simulink library "Model_DG_Synchronous_Generator"  (R2022b)
settings: Solver=VariableStepAuto  StartTime=0.0  StopTime=10.0  RelTol=1e-3
libraries: eeGeneralControl x11, simulink x6, slpidlib x4, spsPositiveSequencePLLDrivenLib x3, spsAC1AExcitationSystemLib x1, spsAC4AExcitationSystemLib x1, spsAC5AExcitationSystemLib x1, spsDC1AExcitationSystemLib x1, spsDC2AExcitationSystemLib x1, spsST1AExcitationSystemLib x1, spsST2AExcitationSystemLib x1, spsPLL3phLib x1
(part 1 of 2)
settings Model: Creator=winkens  LastModifiedBy=winkens
settings SolverCC: AlgebraicLoopSolver=TrustRegion
settings DebuggingCC: UnconnectedInputMsg=warning  UnconnectedOutputMsg=warning  UnconnectedLineMsg=warning  SFMachineParentedDataDiag=warning
settings ModelReferenceCC: EnableRefExpFcnMdlSchedulingChecks=on
settings RTWCC: DLArmComputeVersion=19.05

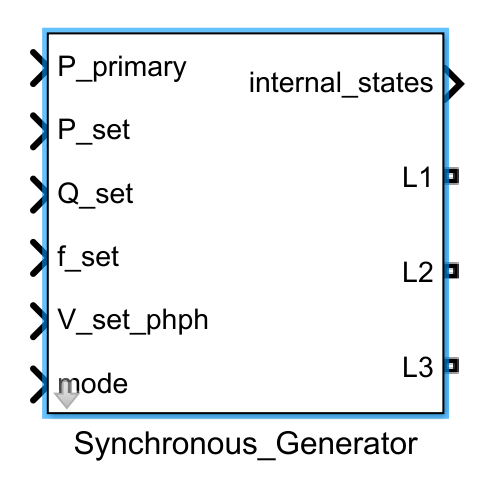
[thumbnail: Simulink's stored preview of the top-level diagram]
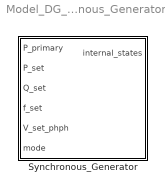
== system Model_DG_Synchronous_Generator ==
  Synchronous_Generator : Subsystem  mask{S_n=3.2e6, P_binst=2.0e6, V_n_phph=400, V_n_grid_phph=20e3, f_n=50, T_s_ctrl=1e-4, T_s_meas=1e-4, datatype='double', SG_Reactances=[ 3.19 0.33 0.159 1.79 0.155 0.05 ], SG_TimeConstants=[ 0.5 0.025 0.025 ], SG_StatorResistance=0.00074, SG_mech=[ 0.366 0.01 2 ], gov_type=IEEEG1 simplified, K_IEEEG1simp=10, T_IEEEG1simp=[ 0.2 0 0.1 0 ], dP_maxmin_IEEEG1simp=[ 2 -2 ], K_TGOV1=20, T_TGOV1=[ 0.2 0.6 2 ], kd_TGOV1=0.05, exciterModel=AC1A, QCtrl=Constant Voltage (no Q-Control), K_p_QCtrl=0.5, K_i_QCtrl=0.4, uq0ref=1.0, qmax=0.33, umax=1.04, deadband=0, p_pu=[0.1, 0.5, 0.6, 0.9, 1.0], q_pu=[0.0, 0.0, -0.05, -0.33, -0.33], p1=[0.94, 0.33], p2=[0.96, 0], p3=[1.04, 0], p4=[1.06, -0.33], cosphi_ref=1, ind_cap_Q=Inductive behavior (capacitive Q infeed), use_transformer=Grid coupling with transformer, RL_Trafo_GenSide=[ 0.002 0.08 ], RL_Trafo_GridSide=[ 0.002 0.08 ], Trafo_RmLm=[ 500 500 ]}
      mask prompts: S_n "Nominal Apparent Power [VA]"; P_binst "Installed Active Power [W]"; V_n_phph "Nominal Generator Voltage (rms, phase-to-phase) [V]"; V_n_grid_phph "Nominal Grid Voltage (rms, phase-to-phase) [V]"; f_n "Nominal Frequency [Hz]"; T_s_ctrl "Controller sample time [s]"; T_s_meas "Measurement sample time [s]"; datatype "Signal data type"; SG_Reactances "Reactances [ Xd Xd' Xd'' Xq Xq'' Xl ] (pu)"; SG_TimeConstants "Time constants [ Td' Td'' Tq'' ]  (s)"; SG_StatorResistance "Stator resistance (pu)"; SG_mech "Inertia, friction factor, pole pairs [ H(s) F(pu) p ]"; gov_type "Type"; K_IEEEG1simp "Droop Gain dP/df (pu)"; T_IEEEG1simp "Time Constants [ T1 T2 T3 T4 ] (s)"; dP_maxmin_IEEEG1simp "Max. rate of change of mech. power [ dP_max dP_min ] (pu)"; K_TGOV1 "Droop Gain dP/df (pu)"; T_TGOV1 "Time Constants [ T1 T2 T3 ] (s)"; kd_TGOV1 "Max. rate of change of mech. power [ dP_max dP_min ] (pu)"; exciterModel "Exciter Type"; QCtrl "Mode"; K_p_QCtrl "Q-Controller Proportional Gain"; K_i_QCtrl "Q-Controller Integral Gain"; uq0ref "U_Q0ref [pu]"; qmax "|Q_max| [pu]"; umax "U_max [pu]"; deadband "Voltage Deadband [+- %]"; p_pu "P_grid points [pu]"; q_pu "Q_grid points [pu]"; p1 "P1 [V_grid, Q_grid] [pu]"; p2 "P2 [V_grid, Q_grid] [pu]"; p3 "P3 [V_grid, Q_grid] [pu]"; p4 "P4 [V_grid, Q_grid] [pu]"; cosphi_ref "cos(phi)"; use_transformer "Transformer usage"; RL_Trafo_GenSide "SG-side winding impedance [ R L ] (pu):"; RL_Trafo_GridSide "Grid-side winding impedance [ R L ] (pu):"; Trafo_RmLm "Magnetization resistance and inductance [ Rm(pu) Lm(pu) ]"
      mask init:
      | alpha1 = (2*T_TGOV1(1)-T_s_ctrl) / (2*T_TGOV1(1)+T_s_ctrl);
      |     alpha2 = (2*T_TGOV1(2)-T_s_ctrl) / (2*T_TGOV1(2)+T_s_ctrl);
      |     alpha3 = (2*T_TGOV1(3)-T_s_ctrl) / (2*T_TGOV1(3)+T_s_ctrl);
      mask TypeOptions gov_type: IEEEG1 simplified | GAST (Generator Test Bench at Distribution Grid Laboratory) | TGOV1
      mask TypeOptions exciterModel: AC1A | AC4A | AC5A | DC1A | DC2A | ST1A | ST2A | AVR_Huette
      mask Callback exciterModel:
      | if strcmp(get_param(gcb,'exciterModel'),'AC1A')
      |     set_param([gcb '/SG_Control/Exciter'],'LabelModeActivechoice','AC1A');
      | 
      | elseif strcmp(get_param(gcb,'exciterModel'),'AC4A')
      |     set_param([gcb '/SG_Control/Exciter'],'LabelModeActivechoice','AC4A');
      | 
      | elseif strcmp(get_param(gcb,'exciterModel'),'AC5A')
      |     set_param([gcb '/SG_Control/Exciter'],'LabelModeActivechoice','AC5A');
      | 
      | elseif strcmp(get_param(gcb,'exciterModel'),'DC1A')
      |     set_param([gcb '/SG_Control/Exciter'],'LabelModeActivechoice','DC1A');
      | 
      | elseif strcmp(get_param(gcb,'exciterModel'),'DC2A')
      |     set_param([gcb '/SG_Control/Exciter'],'LabelModeActivechoice','DC2A');
      | 
      | elseif strcmp(get_param(gcb,'exciterModel'),'ST1A')
      |     set_param([gcb '/SG_Control/Exciter'],'LabelModeActivechoice','ST1A');
      | 
      | elseif strcmp(get_param(gcb,'exciterModel'),'ST2A')
      |     set_param([gcb '/SG_Control/Exciter'],'LabelModeActivechoice','ST2A');
      | 
      | elseif strcmp(get_param(gcb,'exciterModel'),'AVR_Huette')
      |     set_param([gcb '/SG_Control/Exciter'],'LabelModeActivechoice','AVR_Huette');
      | 
      | else
      |     set_param([gcb '/SG_Control/Exciter'],'LabelModeActivechoice','DC1A');
      | 
      | end
      mask TypeOptions QCtrl: Constant Voltage (no Q-Control) | Q(V)-Curve | Q(P)-Curve | Constant Q with Q(V)-Limitation | Constant cos(phi)
      mask Callback QCtrl:
      | msk = Simulink.Mask.get(gcb);
      | if strcmp(get_param(gcb,'QCtrl'),'Q(V)-Curve')
      |     %(a) Q(V)
      |     msk.getDialogControl('parambox_QV').Visible = 'on';
      |     msk.getDialogControl('parambox_QP').Visible = 'off';
      |     msk.getDialogControl('parambox_constQ').Visible = 'off';
      |     msk.getDialogControl('parambox_cosphi').Visible = 'off';
      | 
      | elseif strcmp(get_param(gcb,'QCtrl'),'Q(P)-Curve')
      |     %(b) Q(P)
      |     msk.getDialogControl('parambox_QV').Visible = 'off';
      |     msk.getDialogControl('parambox_QP').Visible = 'on';
      |     msk.getDialogControl('parambox_constQ').Visible = 'off';
      |     msk.getDialogControl('parambox_cosphi').Visible = 'off';
      | 
      | elseif strcmp(get_param(gcb,'QCtrl'),'Constant Q with Q(V)-Limitation')
      |     %(c) const Q
      |     msk.getDialogControl('parambox_QV').Visible = 'off';
      |     msk.getDialogControl('parambox_QP').Visible = 'off';
      |     msk.getDialogControl('parambox_constQ').Visible = 'on';
      |     msk.getDialogControl('parambox_cosphi').Visible = 'off';
      | 
      | elseif strcmp(get_param(gcb,'QCtrl'),'Constant cos(phi)')
      |     %(d) const cosphi
      |     msk.getDialogControl('parambox_QV').Visible = 'off';
      |     msk.getDialogControl('parambox_QP').Visible = 'off';
      |     msk.getDialogControl('parambox_constQ').Visible = 'off';
      |     msk.getDialogControl('parambox_cosphi').Visible = 'on';
      | 
      | elseif strcmp(get_param(gcb,'QCtrl'),'Constant Voltage (no Q-Control)')
      |     % no Q-Control
      |     msk.getDialogControl('parambox_QV').Visible = 'off';
      |     msk.getDialogControl('parambox_QP').Visible = 'off';
      |     msk.getDialogControl('parambox_constQ').Visible = 'off';
      |     msk.getDialogControl('parambox_cosphi').Visible = 'off';
      | 
      | end
      mask TypeOptions ind_cap_Q: Inductive behavior (capacitive Q infeed) | Capacitive behavior (inductive Q infeed)
      mask TypeOptions use_transformer: Direct grid coupling of SG (without transformer) | Grid coupling with transformer
      mask DialogControl DescGroupVar Prompt: Synchronous Generator
      mask DialogControl DescTextVar Prompt: Distributed generation unit using a synchronous generator for electromechanical energy conversion.
      mask DialogControl Container4 Prompt: General
      mask DialogControl Container24 Prompt: Sample Times and Data Types
      mask DialogControl Container5 Prompt: Synchr. Gen.
      mask DialogControl Control2 Prompt: All Synchronous Generator Parameters are defined in a per-unit-system based on the nominal apparent power, nominal generator voltage and nominal frequency defined in general-tab.
      mask DialogControl Container11 Prompt: Parameters
      mask DialogControl Container6 Prompt: Governor
      mask DialogControl Container13 Prompt: Parameters (Simplified IEEEG1-Governor-Turbine-Model)
      mask DialogControl Container13_copy Prompt: Parameters (TGOV1)
      mask DialogControl Container7 Prompt: Exciter
      mask DialogControl Container8 Prompt: Q-Control
      mask DialogControl Control3 Prompt: Reactive power control according to German MV grid codes VDE 4110. Choose constant voltage mode for no reactive power control in grid-forming units.
      mask DialogControl Container17 Prompt: Parameters
      mask DialogControl parambox_QV Prompt: Q(V) Parameters
      mask DialogControl parambox_QP Prompt: Q(P) Parameters
      mask DialogControl parambox_constQ Prompt: Constant Q with Q(V)-Limitation Parameters
      mask DialogControl parambox_cosphi Prompt: Constant cos(phi) Parameters
      mask DialogControl Container10 Prompt: Transformer
      mask DialogControl Control4 Prompt: Transformer parameters are defined in a per-unit-system based on the nominal power, the nominal frequency and the nominal voltages defined in tab General. The reference voltage for the impedance values depends on the respective nominal voltage level. However, magnetization resistance and inductance are based on the generator-side nominal voltage.
      mask DialogControl Container20 Prompt: Parameters

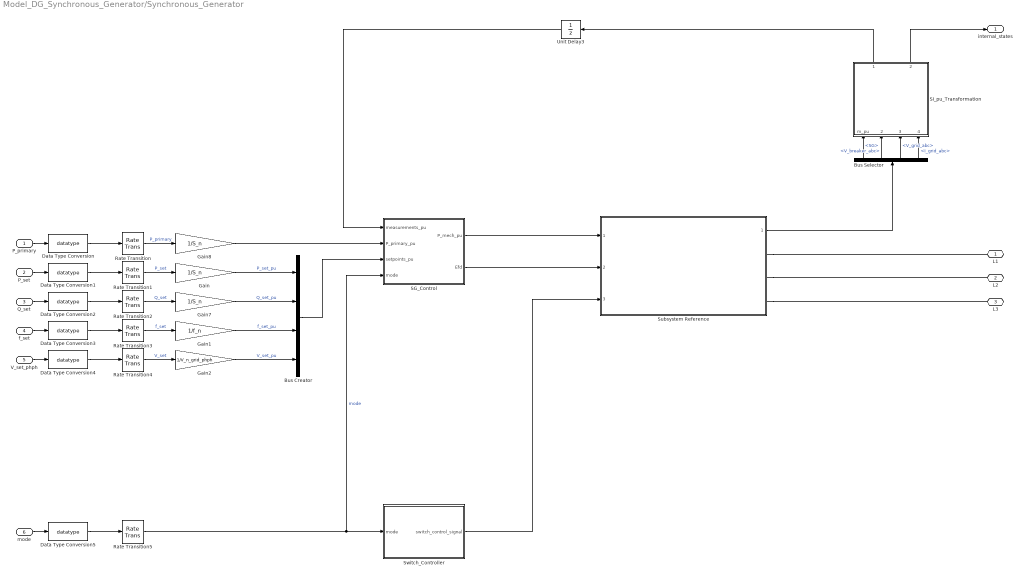
== system Model_DG_Synchronous_Generator/Synchronous_Generator ==
  P_primary : Inport
  P_set : Inport  Port=2
  Q_set : Inport  Port=3
  f_set : Inport  Port=4
  V_set_phph : Inport  Port=5
  mode : Inport  Port=6
  Bus Creator : BusCreator  Inputs=4
  Bus Selector : BusSelector  OutputSignals=SG,V_breaker_abc,V_grid_abc,I_grid_abc
  Data Type Conversion{,1..5} (6 alike) : DataTypeConversion  OutDataTypeStr=datatype  SaturateOnIntegerOverflow=off  RndMeth=Floor
  Gain : Gain  Gain=1/S_n
  Gain1 : Gain  Gain=1/f_n
  Gain2 : Gain  Gain=1/V_n_grid_phph
  Gain7 : Gain  Gain=1/S_n
  Gain8 : Gain  Gain=1/S_n
  Rate Transition{,1..5} (6 alike) : RateTransition  OutPortSampleTime=T_s_ctrl
  SG_Control : Subsystem
  SI_pu_Transformation : Subsystem
  Subsystem Reference : Subsystem  ReferencedSubsystem=Subsys_SG_Electromechanical_Part_SPS  S_n=S_n  f_n=f_n  V_n_phph=V_n_phph  V_n_grid_phph=V_n_grid_phph  SG_Reactances=SG_Reactances  SG_TimeConstants=SG_TimeConstants  SG_StatorResistance=SG_StatorResistance  SG_mech=SG_mech  use_transformer=use_transformer - 1  RL_Trafo_GenSide=RL_Trafo_GenSide  RL_Trafo_GridSide=RL_Trafo_GridSide  Rm_Lm=Trafo_RmLm  T_s_meas=T_s_meas  datatype=datatype
  Switch_Controller : Subsystem
  Unit Delay3 : UnitDelay  SampleTime=-1  HasFrameUpgradeWarning=on
  L1 : PMIOPort  Side=Right
  L2 : PMIOPort  Port=2  Side=Right
  L3 : PMIOPort  Port=3  Side=Right
  internal_states : Outport
  wires:
  V_set_phph/1 -> Data Type Conversion4/1
  P_set/1 -> Data Type Conversion1/1
  f_set/1 -> Data Type Conversion3/1
  SI_pu_Transformation/2(measurements_SI) -> internal_states/1
  SI_pu_Transformation/1(measurements_pu) -> Unit Delay3/1
  Q_set/1 -> Data Type Conversion2/1
  P_primary/1 -> Data Type Conversion/1
  Gain/1 -> Bus Creator/1  "P_set_pu"
  Gain7/1 -> Bus Creator/2  "Q_set_pu"
  Gain1/1 -> Bus Creator/3  "f_set_pu"
  Gain2/1 -> Bus Creator/4  "V_set_pu"
  SG_Control/1(P_mech_pu) -> Subsystem Reference/1
  SG_Control/2(Efd) -> Subsystem Reference/2
  Gain8/1 -> SG_Control/2(P_primary_pu)
  Bus Creator/1 -> SG_Control/3(setpoints_pu)
  Unit Delay3/1 -> SG_Control/1(measurements_pu)
  Data Type Conversion5/1 -> Rate Transition5/1
  Switch_Controller/1(switch_control_signal) -> Subsystem Reference/3
  Subsystem Reference/1 -> Bus Selector/1
  Bus Selector/1 -> SI_pu_Transformation/1(m_pu)  "<SG>"
  Bus Selector/2 -> SI_pu_Transformation/2(V_breaker_SI)  "<V_breaker_abc>"
  Bus Selector/3 -> SI_pu_Transformation/3(V_grid_SI)  "<V_grid_abc>"
  Bus Selector/4 -> SI_pu_Transformation/4(I_grid_SI)  "<I_grid_abc>"
  Data Type Conversion/1 -> Rate Transition/1
  Data Type Conversion1/1 -> Rate Transition1/1
  Data Type Conversion2/1 -> Rate Transition2/1
  Data Type Conversion3/1 -> Rate Transition3/1
  Data Type Conversion4/1 -> Rate Transition4/1
  mode/1 -> Data Type Conversion5/1
  Rate Transition/1 -> Gain8/1  "P_primary"
  Rate Transition1/1 -> Gain/1  "P_set"
  Rate Transition2/1 -> Gain7/1  "Q_set"
  Rate Transition3/1 -> Gain1/1  "f_set"
  Rate Transition4/1 -> Gain2/1  "V_set"
  Rate Transition5/1 -> SG_Control/4(mode), Switch_Controller/1(mode)  "mode"
  connections:
  Subsystem Reference/RConn2 -- L2/RConn1
  Subsystem Reference/RConn1 -- L1/RConn1
  Subsystem Reference/RConn3 -- L3/RConn1

== system Model_DG_Synchronous_Generator/Synchronous_Generator/SG_Control ==
  note: Speed Control
  note: Voltage Control
  note: Measurements and Setpoints
  measurements_pu : Inport
  P_primary_pu : Inport  Port=2
  setpoints_pu : Inport  Port=3
  mode : Inport  Port=4
  Bus Selector : BusSelector  OutputSignals="electrical_pu.V_breaker_rms_posSeq_pu,electrical_pu.V_grid_rms_posSeq_pu,SG_pu.Mechanical.Rotor speed  wm  (pu),electrical_pu.I_grid_pu,SG_pu.dq0 components.Field current  ifd (pu),electrical_pu.P_grid_pu,electrical_pu.Q_grid_pu,electrical_pu.V_grid_phase_posSeq,electrical_pu.V_breaker_phase_posSeq,electrical_pu.f_grid_PLL_pu"
  Bus Selector1 : BusSelector  OutputSignals=V_set_pu,f_set_pu,P_set_pu,Q_set_pu
  Exciter : Subsystem  Variant=on  VariantControlMode=label  LabelModeActiveChoice=AC1A
      settings: AttributesFormatString=%<BlockChoice>
  Governor_and_Turbine : Subsystem  Variant=on
  Multiport Switch : MultiPortSwitch  Inputs=2  DiagnosticForDefault=None  SaturateOnIntegerOverflow=off  InputSameDT=off
  Reactive_Power_Controller : Subsystem  Variant=on
  Synchronization_Controller : Subsystem
  P_mech_pu : Outport
  Efd : Outport  Port=2
  wires:
  Exciter/1(Efd) -> Efd/1
  Governor_and_Turbine/1(P_mech_pu) -> P_mech_pu/1
  Reactive_Power_Controller/1(V_stab_pu) -> Exciter/5(Vstab)
  measurements_pu/1 -> Bus Selector/1
  setpoints_pu/1 -> Bus Selector1/1
  Bus Selector1/3 -> Governor_and_Turbine/4(P_ref_pu)  "<P_set_pu>"
  Bus Selector/3 -> Governor_and_Turbine/3(omega_pu)  "<Rotor speed  wm  (pu)>"
  P_primary_pu/1 -> Governor_and_Turbine/5(P_primary_pu)
  Multiport Switch/1 -> Reactive_Power_Controller/2(V_grid_pu), Exciter/2(Vt)
  Bus Selector/4 -> Exciter/3(It)  "<I_grid_pu>"
  Bus Selector/5 -> Exciter/4(Ifd)  "<Field current  ifd (pu)>"
  mode/1 -> Multiport Switch/1, Governor_and_Turbine/1(mode), Reactive_Power_Controller/1(mode), Synchronization_Controller/1(mode)
  Bus Selector1/4 -> Reactive_Power_Controller/3(Q_set_pu)  "<Q_set_pu>"
  Bus Selector/2 -> Synchronization_Controller/4(V_grid_posSeq_pu), Multiport Switch/3  "<V_grid_rms_posSeq_pu>"
  Bus Selector/1 -> Multiport Switch/2  "<V_breaker_rms_posSeq_pu>"
  Bus Selector/6 -> Reactive_Power_Controller/4(P_grid_pu)  "<P_grid_pu>"
  Bus Selector/7 -> Reactive_Power_Controller/5(Q_grid_pu)  "<Q_grid_pu>"
  Synchronization_Controller/2(omega_ref_pu) -> Governor_and_Turbine/2(omega_ref_pu)
  Synchronization_Controller/1(V_ref_pu) -> Exciter/1(Vref)
  Bus Selector1/1 -> Synchronization_Controller/2(V_set_pu)  "<V_set_pu>"
  Bus Selector1/2 -> Synchronization_Controller/3(f_set_pu)  "<f_set_pu>"
  Bus Selector/8 -> Synchronization_Controller/5(theta_grid_posSeq)  "<V_grid_phase_posSeq>"
  Bus Selector/9 -> Synchronization_Controller/6(theta_breaker_posSeq)  "<V_breaker_phase_posSeq>"
  Bus Selector/10 -> Synchronization_Controller/7(f_grid_pu)  "<f_grid_PLL_pu>"

== system Model_DG_Synchronous_Generator/Synchronous_Generator/SI_pu_Transformation ==
  m_pu : Inport
  V_breaker_SI : Inport  Port=2
  V_grid_SI : Inport  Port=3
  I_grid_SI : Inport  Port=4
  Bus Creator : BusCreator  Inputs=11
  Bus Creator1 : BusCreator  Inputs=2
  Bus Creator2 : BusCreator  Inputs=2
  Electrical_Measurements_To_pu : Subsystem
  Positive_Sequence_Calculation : Subsystem
  SG_Measurements_To_SI : Subsystem
  measurements_pu : Outport
  measurements_SI : Outport  Port=2
  wires:
  m_pu/1 -> Bus Creator2/1, SG_Measurements_To_SI/1(m_pu)  "SG_pu"
  V_breaker_SI/1 -> Positive_Sequence_Calculation/2(V_breaker_abc), Bus Creator/1  "V_breaker_SI"
  V_grid_SI/1 -> Positive_Sequence_Calculation/1(V_grid_abc), Bus Creator/2  "V_grid_SI"
  I_grid_SI/1 -> Positive_Sequence_Calculation/3(I_grid_abc), Bus Creator/3  "I_grid_SI"
  Bus Creator/1 -> Bus Creator1/2, Electrical_Measurements_To_pu/1(el_SI)  "electrical_SI"
  Bus Creator1/1 -> measurements_SI/1
  Bus Creator2/1 -> measurements_pu/1
  Electrical_Measurements_To_pu/1(el_pu) -> Bus Creator2/2  "electrical_pu"
  SG_Measurements_To_SI/1(m_SI) -> Bus Creator1/1  "SG_SI"
  Positive_Sequence_Calculation/1(P_grid_SI) -> Bus Creator/4  "P_grid_SI"
  Positive_Sequence_Calculation/2(Q_grid_SI) -> Bus Creator/5  "Q_grid_SI"
  Positive_Sequence_Calculation/3(V_grid_rms_posSeq_SI) -> Bus Creator/6  "V_grid_rms_posSeq_SI"
  Positive_Sequence_Calculation/4(I_grid_rms_posSeq_SI) -> Bus Creator/7  "I_grid_rms_posSeq_SI"
  Positive_Sequence_Calculation/5(V_breaker_rms_posSeq_SI) -> Bus Creator/8  "V_breaker_rms_posSeq_SI"
  Positive_Sequence_Calculation/6(V_grid_phase_posSeq_SI) -> Bus Creator/9  "V_grid_phase_posSeq"
  Positive_Sequence_Calculation/7(V_breaker_phase_posSeq_SI) -> Bus Creator/10  "V_breaker_phase_posSeq"
  Positive_Sequence_Calculation/8(f_grid_PLL_SI) -> Bus Creator/11  "f_grid_PLL_SI"

== system Model_DG_Synchronous_Generator/Synchronous_Generator/Switch_Controller ==
  note: Blackstart
  note: Synchronization
  note: Grid Parallel Operation
  mode : Inport
  Constant{,1..3} (4 alike) : Constant
  Constant4 : Constant  Value=0
  Constant5 : Constant  Value=0
  Multiport Switch : MultiPortSwitch  DataPortOrder=Zero-based contiguous  zeroidx=on  SaturateOnIntegerOverflow=off  InputSameDT=off
  Mux : Mux  Inputs=2
  Mux1 : Mux  Inputs=2
  Mux2 : Mux  Inputs=2
  switch_control_signal : Outport
  wires:
  mode/1 -> Multiport Switch/1
  Multiport Switch/1 -> switch_control_signal/1
  Mux/1 -> Multiport Switch/2
  Mux2/1 -> Multiport Switch/4
  Mux1/1 -> Multiport Switch/3
  Constant/1 -> Mux/1
  Constant1/1 -> Mux/2
  Constant2/1 -> Mux2/1
  Constant3/1 -> Mux1/2
  Constant4/1 -> Mux1/1
  Constant5/1 -> Mux2/2

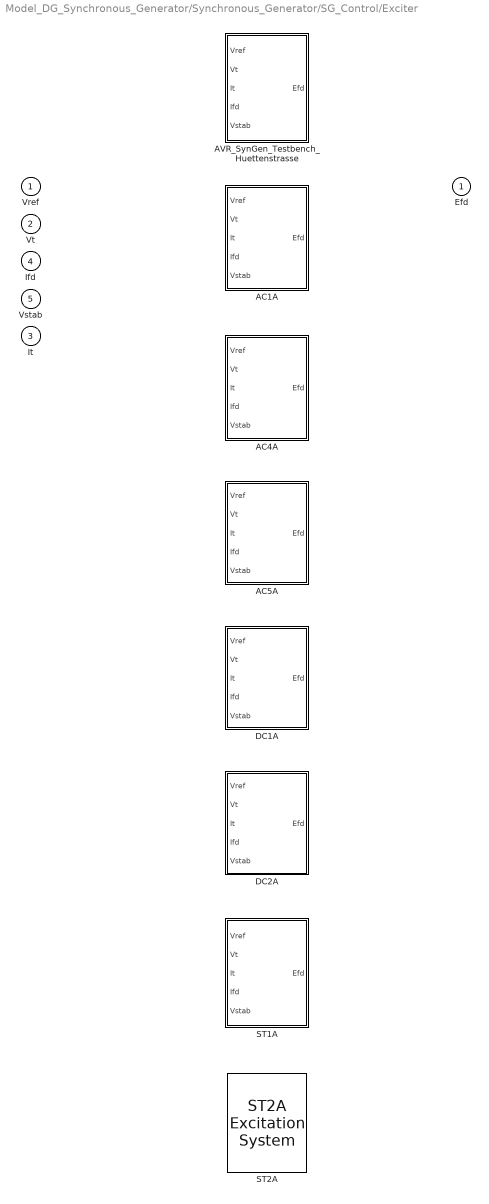
== system Model_DG_Synchronous_Generator/Synchronous_Generator/SG_Control/Exciter ==
  Vref : Inport
  Vt : Inport  Port=2
  It : Inport  Port=3
  Ifd : Inport  Port=4
  Vstab : Inport  Port=5
  AC1A : Subsystem  VariantControl=AC1A
  AC4A : Subsystem  VariantControl=AC4A
  AC5A : Subsystem  VariantControl=AC5A
  AVR_SynGen_Testbench_Huettenstrasse : Subsystem  VariantControl=AVR_Huette
  DC1A : Subsystem  VariantControl=DC1A
  DC2A : Subsystem  VariantControl=DC2A
  ST1A : Subsystem  VariantControl=ST1A
  ST2A : spsST2AExcitationSystemLib/ST2A Excitation System  VariantControl=ST2A  Tr=20e-3  KaTa=[120 0.15]  VRminmax=[0 1.0]  KfTf=[0.05 1.0]  KeTe=[1.0 0.5]  KI=0  Kp=4.88  Xd=1.56  Kc=0.1  v0=[1,1.42734]  I0=0.2739  TsBlock=-2
  Efd : Outport  VectorParamsAs1DForOutWhenUnconnected=off

== system Model_DG_Synchronous_Generator/Synchronous_Generator/SG_Control/Governor_and_Turbine ==
  note: 1) Add Subsystem or Model blocks as valid variant choices.
      | 2) You cannot connect blocks at this level. At simulation, connectivity is automatically
      | determined, based on the active variant and port name matching.
  mode : Inport
  omega_ref_pu : Inport  Port=2
  omega_pu : Inport  Port=3
  P_ref_pu : Inport  Port=4
  P_primary_pu : Inport  Port=5
  GAST_SyncGen_Testbench_Huettenstrasse : Subsystem  VariantControl=gov_type == 2
  IEEEG1_simplified : Subsystem  VariantControl=(default)
  TGOV1 : Subsystem  VariantControl=gov_type > 2.5
  P_mech_pu : Outport

== system Model_DG_Synchronous_Generator/Synchronous_Generator/SG_Control/Reactive_Power_Controller ==
  note: 1) Add Subsystem or Model blocks as valid variant choices.
      | 2) You cannot connect blocks at this level. At simulation, connectivity is automatically
      | determined, based on the active variant and port name matching.
  mode : Inport
  V_grid_pu : Inport  Port=2
  Q_set_pu : Inport  Port=3
  P_grid_pu : Inport  Port=4
  Q_grid_pu : Inport  Port=5
  Constant_Voltage : Subsystem  VariantControl=(default)
  Reactive_Power_Control : Subsystem  VariantControl=QCtrl > 1.5
  V_stab_pu : Outport

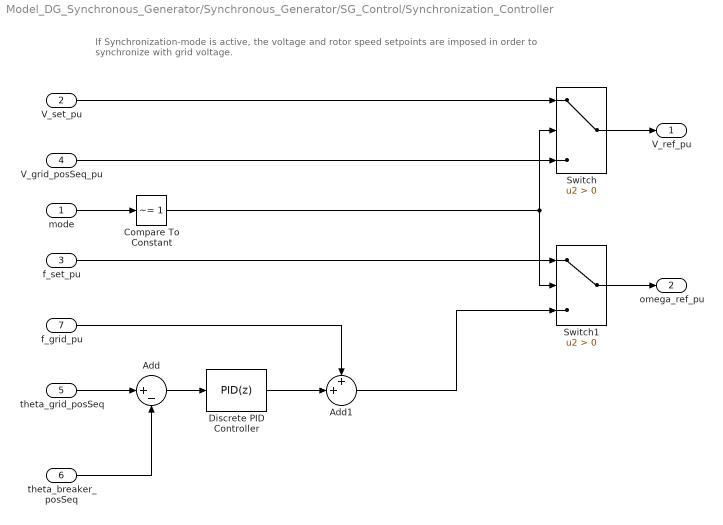
== system Model_DG_Synchronous_Generator/Synchronous_Generator/SG_Control/Synchronization_Controller ==
  note: If Synchronization-mode is active, the voltage and rotor speed setpoints are imposed in order to synchronize with grid voltage.
  mode : Inport
  V_set_pu : Inport  Port=2
  f_set_pu : Inport  Port=3
  V_grid_posSeq_pu : Inport  Port=4
  theta_grid_posSeq : Inport  Port=5
  theta_breaker_posSeq : Inport  Port=6
  f_grid_pu : Inport  Port=7
  Add : Sum  Inputs=|+-
  Add1 : Sum  Inputs=++|
  Compare To Constant : simulink/Logic and Bit Operations/Compare To Constant  relop=~=  const=1  OutDataTypeStr=boolean
  Discrete PID Controller : slpidlib/PID Controller  Controller=PID  Form=Parallel  TimeDomain=Discrete-time  UseExternalTs=off  SampleTime=-1  IntegratorMethod=Forward Euler  FilterMethod=Forward Euler  ControllerParametersSource=internal  P=0.01  I=0.01  UseKiTs=off  D=0.01  N=100  UseFilter=on  TunerSelectOption=Transfer Function Based (PID Tuner App)  InitialConditionSource=internal  InitialConditionForIntegrator=0  InitialConditionForFilter=0  DifferentiatorICPrevScaledInput=0  ExternalReset=none  TrackingMode=off  Kt=1  LimitOutput=on  SatLimitsSource=internal  UpperSaturationLimit=0.005  LowerSaturationLimit=-0.005  LinearizeAsGain=off  AntiWindupMode=clamping  Kb=1  LimitIntegrator=off  UpperIntegratorSaturationLimit=inf  LowerIntegratorSaturationLimit=-inf  POutMin=[]  POutMax=[]  IOutMin=[]  IOutMax=[]  DOutMin=[]  DOutMax=[]  NOutMin=[]  NOutMax=[]  SumOutMin=[]  SumOutMax=[]  SaturationOutMin=[]  SaturationOutMax=[]  PParamMin=[]  PParamMax=[]  IParamMin=[]  IParamMax=[]  DParamMin=[]  DParamMax=[]  NParamMin=[]  NParamMax=[]  KbParamMin=[]  KbParamMax=[]  KtParamMin=[]  KtParamMax=[]  KbOutMin=[]  KbOutMax=[]  KtOutMin=[]  KtOutMax=[]  IntegratorOutMin=[]  IntegratorOutMax=[]  FilterOutMin=[]  FilterOutMax=[]  SumI1OutMin=[]  SumI1OutMax=[]  SumI2OutMin=[]  SumI2OutMax=[]  SumI3OutMin=[]  SumI3OutMax=[]  SumI4OutMin=[]  SumI4OutMax=[]  SumDOutMin=[]  SumDOutMax=[]  DifferentiatorOutMin=[]  DifferentiatorOutMax=[]  FilterDiffOutCoefMin=[]  FilterDiffOutCoefMax=[]  ReciprocalOutMin=[]  ReciprocalOutMax=[]  SumDenOutMin=[]  SumDenOutMax=[]  SumNumOutMin=[]  SumNumOutMax=[]  DivideOutMin=[]  DivideOutMax=[]  UdiffTsProdOutMin=[]  UdiffTsProdOutMax=[]  NTsProdOutMin=[]  NTsProdOutMax=[]  UintegralTsProdOutMin=[]  UintegralTsProdOutMax=[]  UngainTsProdOutMin=[]  UngainTsProdOutMax=[]  ClampingZeroOutDataTypeStr=Inherit: Inherit via back propagation  ClampingZeroOutMin=[]  ClampingZeroOutMax=[]  FilterDenConstantOutDataTypeStr=Inherit: Inherit via back propagation  FilterDenConstantOutMin=[]  FilterDenConstantOutMax=[]  PCopyOutDataTypeStr=Inherit: Inherit via back propagation  PCopyOutMin=[]  PCopyOutMax=[]  NCopyOutDataTypeStr=Inherit: Inherit via back propagation  NCopyOutMin=[]  NCopyOutMax=[]  IntegratorContinuousStateAttributes=''  IntegratorStateMustResolveToSignalObject=off  IntegratorRTWStateStorageClass=Auto  FilterContinuousStateAttributes=''  FilterStateMustResolveToSignalObject=off  FilterRTWStateStorageClass=Auto  ParallelPVariant=InternalParameters  IdealPVariant=Disabled  IVariant=InternalParameters  DVariant=InternalParameters  IntegratorVariant=Discrete  SatVariant=Enabled  AWVariant=DiscClampingParallel  PCopyVariant=Disabled  TRVariant=Disabled  FdbkBlocksVariant=Forward  IdealPFdbkVariant=Disabled  SatFdbkVariant=Disabled  DerivativeFilterVariant=ForwardEulerFilter  NVariant=InternalParameters  NCopyVariant=Disabled  FilterICVariant=InternalICsFilter  IntegratorICVariant=InternalICs  ExternalResetVariant=Disabled  TRSumVariant=Passthrough  SumFdbkVariant=Disabled  SumVariant=Sum_PID  TsampFilterVariant=InternalTs  TsampNgainVariant=Passthrough  TsampIntegralVariant=Passthrough  ExternalSaturationOutDataTypeStr=Inherit: Same as second input
  Switch : Switch  Criteria=u2 > Threshold  SaturateOnIntegerOverflow=off  InputSameDT=off
  Switch1 : Switch  Criteria=u2 > Threshold  SaturateOnIntegerOverflow=off  InputSameDT=off
  V_ref_pu : Outport
  omega_ref_pu : Outport  Port=2
  wires:
  mode/1 -> Compare To Constant/1
  Switch/1 -> V_ref_pu/1
  Switch1/1 -> omega_ref_pu/1
  Compare To Constant/1 -> Switch/2, Switch1/2
  f_set_pu/1 -> Switch1/1
  V_set_pu/1 -> Switch/1
  V_grid_posSeq_pu/1 -> Switch/3
  theta_grid_posSeq/1 -> Add/1
  theta_breaker_posSeq/1 -> Add/2
  Add/1 -> Discrete PID Controller/1
  Discrete PID Controller/1 -> Add1/2
  Add1/1 -> Switch1/3
  f_grid_pu/1 -> Add1/1

== system Model_DG_Synchronous_Generator/Synchronous_Generator/SI_pu_Transformation/Electrical_Measurements_To_pu ==
  el_SI : Inport
  Bus Creator : BusCreator  Inputs=11
  Bus Selector : BusSelector  OutputSignals=V_breaker_SI,V_grid_SI,I_grid_SI,P_grid_SI,Q_grid_SI,V_grid_rms_posSeq_SI,I_grid_rms_posSeq_SI,V_breaker_rms_posSeq_SI,V_grid_phase_posSeq,V_breaker_phase_posSeq,f_grid_PLL_SI
  Gain{,1,5,7} (4 alike) : Gain  Gain=sqrt(3)/V_n_grid_phph
  Gain2 : Gain  Gain=(sqrt(3)*V_n_grid_phph) / S_n
  Gain3 : Gain  Gain=1/S_n
  Gain4 : Gain  Gain=1/S_n
  Gain6 : Gain  Gain=(sqrt(3)*V_n_grid_phph) / S_n
  Gain8 : Gain  Gain=1/f_n
  el_pu : Outport
  wires:
  el_SI/1 -> Bus Selector/1
  Bus Selector/1 -> Gain/1  "<V_breaker_SI>"
  Bus Selector/2 -> Gain1/1  "<V_grid_SI>"
  Bus Selector/3 -> Gain2/1  "<I_grid_SI>"
  Gain/1 -> Bus Creator/1  "V_breaker_pu"
  Gain1/1 -> Bus Creator/2  "V_grid_pu"
  Gain2/1 -> Bus Creator/3  "I_grid_pu"
  Bus Creator/1 -> el_pu/1
  Bus Selector/4 -> Gain3/1  "<P_grid_SI>"
  Gain3/1 -> Bus Creator/4  "P_grid_pu"
  Bus Selector/5 -> Gain4/1  "<Q_grid_SI>"
  Gain4/1 -> Bus Creator/5  "Q_grid_pu"
  Bus Selector/6 -> Gain5/1  "<V_grid_rms_posSeq_SI>"
  Gain5/1 -> Bus Creator/6  "V_grid_rms_posSeq_pu"
  Bus Selector/7 -> Gain6/1  "<I_grid_rms_posSeq_SI>"
  Gain6/1 -> Bus Creator/7  "I_grid_rms_posSeq_pu"
  Bus Selector/8 -> Gain7/1  "<V_breaker_rms_posSeq_SI>"
  Gain7/1 -> Bus Creator/8  "V_breaker_rms_posSeq_pu"
  Bus Selector/9 -> Bus Creator/9  "<V_grid_phase_posSeq>"
  Bus Selector/10 -> Bus Creator/10  "<V_breaker_phase_posSeq>"
  Bus Selector/11 -> Gain8/1  "<f_grid_PLL_SI>"
  Gain8/1 -> Bus Creator/11  "f_grid_PLL_pu"

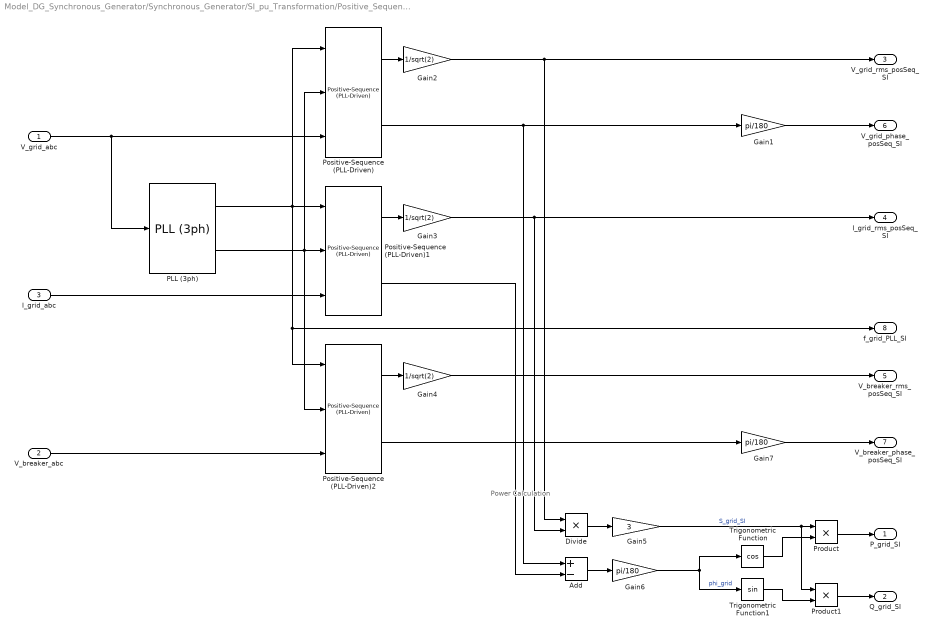
== system Model_DG_Synchronous_Generator/Synchronous_Generator/SI_pu_Transformation/Positive_Sequence_Calculation ==
  note: Power Calculation
  V_grid_abc : Inport
  V_breaker_abc : Inport  Port=2
  I_grid_abc : Inport  Port=3
  Add : Sum  Inputs=+-
  Divide : Product  Inputs=**
  Gain1 : Gain  Gain=pi/180
  Gain2 : Gain  Gain=1/sqrt(2)
  Gain3 : Gain  Gain=1/sqrt(2)
  Gain4 : Gain  Gain=1/sqrt(2)
  Gain5 : Gain  Gain=3
  Gain6 : Gain  Gain=pi/180
  Gain7 : Gain  Gain=pi/180
  PLL (3ph) : spsPLL3phLib/PLL (3ph)  Fmin=35  Par_Init=[0, 50]  ParK=[180, 3200, 1]  TcD=1e-4  MaxRateChangeFreq=12  FilterCutOffFreq=25  Ts=1e-4  AGC=on
  Positive-Sequence (PLL-Driven) : spsPositiveSequencePLLDrivenLib/Positive-Sequence (PLL-Driven)  Finit=50  Fmin=35  InInit=[0, 0]  Ts=T_s_meas
  Positive-Sequence (PLL-Driven)1 : spsPositiveSequencePLLDrivenLib/Positive-Sequence (PLL-Driven)  Finit=50  Fmin=35  InInit=[0, 0]  Ts=T_s_meas
  Positive-Sequence (PLL-Driven)2 : spsPositiveSequencePLLDrivenLib/Positive-Sequence (PLL-Driven)  Finit=50  Fmin=35  InInit=[0, 0]  Ts=T_s_meas
  Product : Product
  Product1 : Product
  Trigonometric Function : Trigonometry  Operator=cos
  Trigonometric Function1 : Trigonometry
  P_grid_SI : Outport
  Q_grid_SI : Outport  Port=2
  V_grid_rms_posSeq_SI : Outport  Port=3
  I_grid_rms_posSeq_SI : Outport  Port=4
  V_breaker_rms_posSeq_SI : Outport  Port=5
  V_grid_phase_posSeq_SI : Outport  Port=6
  V_breaker_phase_posSeq_SI : Outport  Port=7
  f_grid_PLL_SI : Outport  Port=8
  wires:
  V_grid_abc/1 -> PLL (3ph)/1, Positive-Sequence (PLL-Driven)/3
  I_grid_abc/1 -> Positive-Sequence (PLL-Driven)1/3
  V_breaker_abc/1 -> Positive-Sequence (PLL-Driven)2/3
  Positive-Sequence (PLL-Driven)2/1 -> Gain4/1
  Positive-Sequence (PLL-Driven)1/1 -> Gain3/1
  Positive-Sequence (PLL-Driven)/1 -> Gain2/1
  Gain2/1 -> Divide/1, V_grid_rms_posSeq_SI/1
  Gain3/1 -> Divide/2, I_grid_rms_posSeq_SI/1
  Gain4/1 -> V_breaker_rms_posSeq_SI/1
  Divide/1 -> Gain5/1
  Positive-Sequence (PLL-Driven)2/2 -> Gain7/1
  Gain5/1 -> Product1/1, Product/1  "S_grid_SI"
  Positive-Sequence (PLL-Driven)/2 -> Gain1/1, Add/1
  Positive-Sequence (PLL-Driven)1/2 -> Add/2
  Add/1 -> Gain6/1
  Gain6/1 -> Trigonometric Function1/1, Trigonometric Function/1  "phi_grid"
  Product1/1 -> Q_grid_SI/1
  Product/1 -> P_grid_SI/1
  Trigonometric Function/1 -> Product/2
  Trigonometric Function1/1 -> Product1/2
  PLL (3ph)/1 -> Positive-Sequence (PLL-Driven)2/1, f_grid_PLL_SI/1, Positive-Sequence (PLL-Driven)/1, Positive-Sequence (PLL-Driven)1/1
  PLL (3ph)/2 -> Positive-Sequence (PLL-Driven)/2, Positive-Sequence (PLL-Driven)2/2, Positive-Sequence (PLL-Driven)1/2
  Gain1/1 -> V_grid_phase_posSeq_SI/1
  Gain7/1 -> V_breaker_phase_posSeq_SI/1

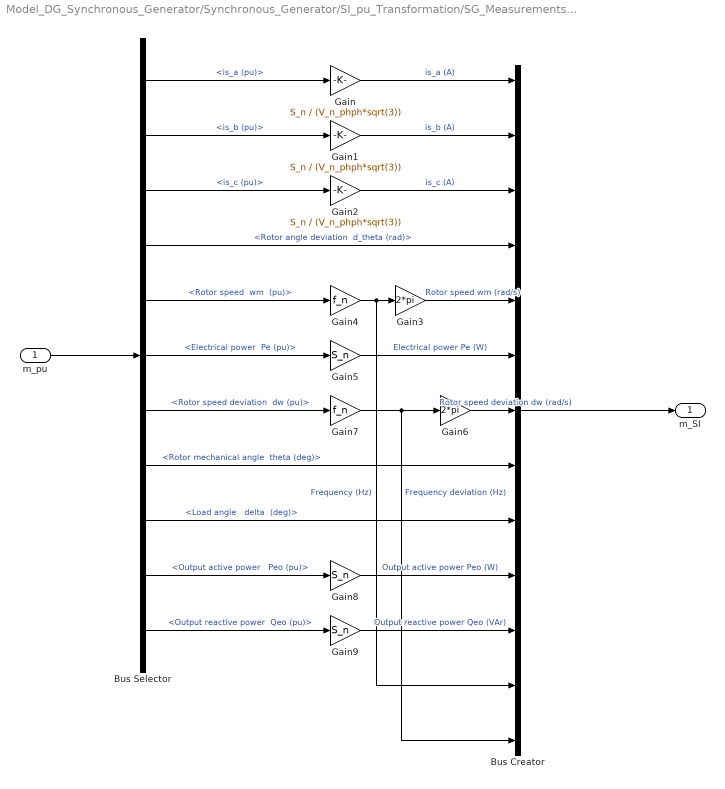
== system Model_DG_Synchronous_Generator/Synchronous_Generator/SI_pu_Transformation/SG_Measurements_To_SI ==
  m_pu : Inport
  Bus Creator : BusCreator  Inputs=13
  Bus Selector : BusSelector  OutputSignals="Stator current.is_a (pu),Stator current.is_b (pu),Stator current.is_c (pu),Mechanical.Rotor angle deviation  d_theta (rad),Mechanical.Rotor speed  wm  (pu),Mechanical.Electrical power  Pe (pu),Mechanical.Rotor speed deviation  dw (pu),Mechanical.Rotor mechanical angle  theta (deg),Load angle   delta  (deg),Output active power   Peo (pu),Output reactive power  Qeo (pu)"
  Gain : Gain  Gain=S_n / (V_n_phph*sqrt(3))
  Gain1 : Gain  Gain=S_n / (V_n_phph*sqrt(3))
  Gain2 : Gain  Gain=S_n / (V_n_phph*sqrt(3))
  Gain3 : Gain  Gain=2*pi
  Gain4 : Gain  Gain=f_n
  Gain5 : Gain  Gain=S_n
  Gain6 : Gain  Gain=2*pi
  Gain7 : Gain  Gain=f_n
  Gain8 : Gain  Gain=S_n
  Gain9 : Gain  Gain=S_n
  m_SI : Outport
  wires:
  m_pu/1 -> Bus Selector/1
  Bus Selector/1 -> Gain/1  "<is_a (pu)>"
  Bus Selector/2 -> Gain1/1  "<is_b (pu)>"
  Bus Selector/3 -> Gain2/1  "<is_c (pu)>"
  Bus Selector/4 -> Bus Creator/4  "<Rotor angle deviation  d_theta (rad)>"
  Bus Selector/5 -> Gain4/1  "<Rotor speed  wm  (pu)>"
  Gain4/1 -> Bus Creator/12, Gain3/1  "Frequency (Hz)"
  Gain3/1 -> Bus Creator/5  "Rotor speed wm (rad/s)"
  Bus Selector/6 -> Gain5/1  "<Electrical power  Pe (pu)>"
  Bus Selector/7 -> Gain7/1  "<Rotor speed deviation  dw (pu)>"
  Gain7/1 -> Gain6/1, Bus Creator/13  "Frequency deviation (Hz)"
  Gain6/1 -> Bus Creator/7  "Rotor speed deviation dw (rad/s)"
  Bus Selector/8 -> Bus Creator/8  "<Rotor mechanical angle  theta (deg)>"
  Bus Selector/9 -> Bus Creator/9  "<Load angle   delta  (deg)>"
  Bus Selector/10 -> Gain8/1  "<Output active power   Peo (pu)>"
  Bus Selector/11 -> Gain9/1  "<Output reactive power  Qeo (pu)>"
  Gain/1 -> Bus Creator/1  "is_a (A)"
  Gain1/1 -> Bus Creator/2  "is_b (A)"
  Gain2/1 -> Bus Creator/3  "is_c (A)"
  Gain5/1 -> Bus Creator/6  "Electrical power Pe (W)"
  Gain8/1 -> Bus Creator/10  "Output active power Peo (W)"
  Gain9/1 -> Bus Creator/11  "Output reactive power Qeo (VAr)"
  Bus Creator/1 -> m_SI/1

== system Model_DG_Synchronous_Generator/Synchronous_Generator/SG_Control/Exciter/AC1A ==
  Vref : Inport
  Vt : Inport  Port=2
  It : Inport  Port=3
  Ifd : Inport  Port=4
  Vstab : Inport  Port=5
  AC1A : spsAC1AExcitationSystemLib/AC1A Excitation System  Tr=20e-3  KaTa=[400 0.02]  VAminmax=[-14.5 14.5]  VRminmax=[-5.43 6.03]  KfTf=[0.03 1.0]  TbTc=[0 0]  KeTe=[1.0 0.80]  Ve12=[4.18 3.14]  SeVe12=[0.10 0.03]  Kd=0.38  Kc=0.20  v0=[0.000416667,0.000461832]*0  TsBlock=-2
  term3 : Terminator
  Efd : Outport  VectorParamsAs1DForOutWhenUnconnected=off
  wires:
  Vref/1 -> AC1A/1
  Vt/1 -> AC1A/2
  Ifd/1 -> AC1A/3
  Vstab/1 -> AC1A/4
  AC1A/1 -> Efd/1
  It/1 -> term3/1

== system Model_DG_Synchronous_Generator/Synchronous_Generator/SG_Control/Exciter/AC4A ==
  Vref : Inport
  Vt : Inport  Port=2
  It : Inport  Port=3
  Ifd : Inport  Port=4
  Vstab : Inport  Port=5
  AC4A : spsAC4AExcitationSystemLib/AC4A Excitation System  Tr=20e-3  KaTa=[200 0.015]  VIminmax=[-10 10]  VRminmax=[-4.53 5.64]  TbTc=[10 1.0]  Kc=0  v0=[1,1.42734]  TsBlock=-2
  term3 : Terminator
  Efd : Outport  VectorParamsAs1DForOutWhenUnconnected=off
  wires:
  Vref/1 -> AC4A/1
  Vt/1 -> AC4A/2
  Ifd/1 -> AC4A/3
  Vstab/1 -> AC4A/4
  AC4A/1 -> Efd/1
  It/1 -> term3/1

== system Model_DG_Synchronous_Generator/Synchronous_Generator/SG_Control/Exciter/AC5A ==
  Vref : Inport
  Vt : Inport  Port=2
  It : Inport  Port=3
  Ifd : Inport  Port=4
  Vstab : Inport  Port=5
  AC5A : spsAC5AExcitationSystemLib/AC5A Excitation System  Tr=20e-3  KaTa=[100 0.02]  VRminmax=[-7.3 7.3]  KfTf=[0.03 1 0 0]  KeTe=[1.0 0.8]  Efd12=[5.6 0.75*5.6]  SeEfd12=[0.86 0.5]  v0=[1,1.42734]  TsBlock=-2
  term3 : Terminator
  term4 : Terminator
  Efd : Outport  VectorParamsAs1DForOutWhenUnconnected=off
  wires:
  Vref/1 -> AC5A/1
  Vt/1 -> AC5A/2
  Vstab/1 -> AC5A/3
  AC5A/1 -> Efd/1
  It/1 -> term3/1
  Ifd/1 -> term4/1

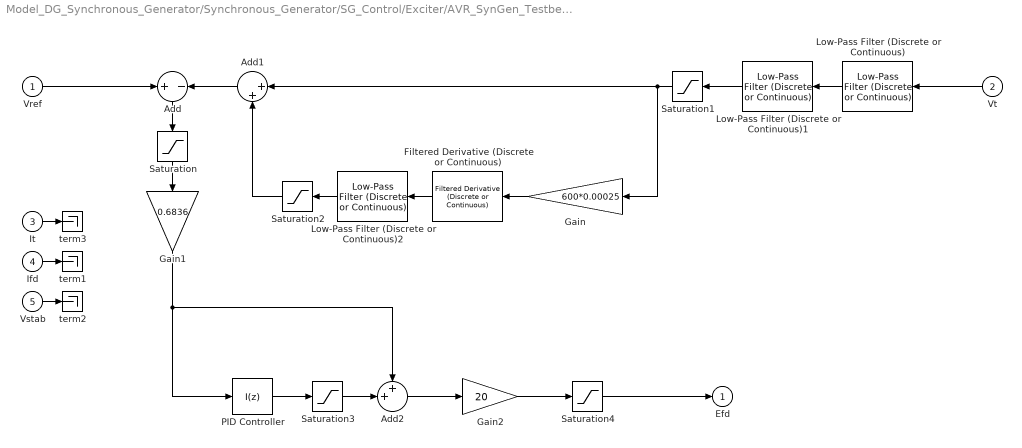
== system Model_DG_Synchronous_Generator/Synchronous_Generator/SG_Control/Exciter/AVR_SynGen_Testbench_Huettenstrasse ==
  Vref : Inport
  Vt : Inport  Port=2
  It : Inport  Port=3
  Ifd : Inport  Port=4
  Vstab : Inport  Port=5
  Add : Sum  Inputs=+|-
  Add1 : Sum  Inputs=|++
  Add2 : Sum  Inputs=++|
  Filtered Derivative (Discrete or Continuous) : eeGeneralControl/Filtered Derivative (Discrete or Continuous)  K=1  T=0.004  B=inf  A=-inf  minRatio=10  init_option=Inherited from block input  x0=0  Ts=-1
  Gain : Gain  Gain=600*0.00025
  Gain1 : Gain  Gain=0.6836
  Gain2 : Gain  Gain=20
  Low-Pass Filter (Discrete or Continuous) : eeGeneralControl/Low-Pass Filter (Discrete or Continuous)  K=1  T=0.002  B=inf  A=-inf  init_option=Inherited from block input  x0=0  Ts=-1
  Low-Pass Filter (Discrete or Continuous)1 : eeGeneralControl/Low-Pass Filter (Discrete or Continuous)  K=1  T=0.0005  B=inf  A=-inf  init_option=Inherited from block input  x0=0  Ts=-1
  Low-Pass Filter (Discrete or Continuous)2 : eeGeneralControl/Low-Pass Filter (Discrete or Continuous)  K=1  T=0.015  B=inf  A=-inf  init_option=Inherited from block input  x0=0  Ts=-1
  PID Controller : slpidlib/PID Controller  Controller=I  Form=Parallel  TimeDomain=Discrete-time  UseExternalTs=off  SampleTime=-1  IntegratorMethod=Forward Euler  FilterMethod=Forward Euler  ControllerParametersSource=internal  P=1  I=1200/131.072  D=0  UseFilter=on  N=100  TunerSelectOption=Transfer Function Based (PID Tuner App)  InitialConditionSource=internal  InitialConditionForIntegrator=0  InitialConditionForFilter=0  DifferentiatorICPrevScaledInput=0  ExternalReset=none  TrackingMode=off  Kt=1  LimitOutput=off  SatLimitsSource=internal  UpperSaturationLimit=inf  LowerSaturationLimit=-inf  LinearizeAsGain=on  AntiWindupMode=none  Kb=1  POutMin=[]  POutMax=[]  IOutMin=[]  IOutMax=[]  DOutMin=[]  DOutMax=[]  NOutMin=[]  NOutMax=[]  SumOutMin=[]  SumOutMax=[]  SaturationOutMin=[]  SaturationOutMax=[]  PParamMin=[]  PParamMax=[]  IParamMin=[]  IParamMax=[]  DParamMin=[]  DParamMax=[]  NParamMin=[]  NParamMax=[]  KbParamMin=[]  KbParamMax=[]  KtParamMin=[]  KtParamMax=[]  KbOutMin=[]  KbOutMax=[]  KtOutMin=[]  KtOutMax=[]  IntegratorOutMin=[]  IntegratorOutMax=[]  FilterOutMin=[]  FilterOutMax=[]  SumI1OutMin=[]  SumI1OutMax=[]  SumI2OutMin=[]  SumI2OutMax=[]  SumI3OutMin=[]  SumI3OutMax=[]  SumI4OutMin=[]  SumI4OutMax=[]  SumDOutMin=[]  SumDOutMax=[]  DifferentiatorOutMin=[]  DifferentiatorOutMax=[]  FilterDiffOutCoefMin=[]  FilterDiffOutCoefMax=[]  ReciprocalOutMin=[]  ReciprocalOutMax=[]  SumDenOutMin=[]  SumDenOutMax=[]  SumNumOutMin=[]  SumNumOutMax=[]  DivideOutMin=[]  DivideOutMax=[]  UdiffTsProdOutMin=[]  UdiffTsProdOutMax=[]  NTsProdOutMin=[]  NTsProdOutMax=[]  UintegralTsProdOutMin=[]  UintegralTsProdOutMax=[]  UngainTsProdOutMin=[]  UngainTsProdOutMax=[]  IntegratorContinuousStateAttributes=''  IntegratorStateMustResolveToSignalObject=off  IntegratorRTWStateStorageClass=Auto  FilterContinuousStateAttributes=''  FilterStateMustResolveToSignalObject=off  FilterRTWStateStorageClass=Auto  ParallelPVariant=Disabled  IdealPVariant=Disabled  IVariant=InternalParameters  DVariant=Disabled  IntegratorVariant=Discrete  SatVariant=Disabled  AWVariant=Passthrough  PCopyVariant=Disabled  TRVariant=Disabled  FdbkBlocksVariant=Forward  IdealPFdbkVariant=Disabled  SatFdbkVariant=Disabled  DerivativeFilterVariant=Disabled  NVariant=Disabled  NCopyVariant=Disabled_SignalSpec  FilterICVariant=Disabled  IntegratorICVariant=InternalICs  ExternalResetVariant=Disabled  TRSumVariant=Passthrough  SumFdbkVariant=Disabled  SumVariant=Passthrough_I  TsampFilterVariant=InternalTs  TsampNgainVariant=Passthrough  TsampIntegralVariant=Passthrough  ExternalSaturationOutDataTypeStr=Inherit: Same as second input
  Saturation : Saturate  UpperLimit=707  LowerLimit=-707
  Saturation1 : Saturate  UpperLimit=707  LowerLimit=-707
  Saturation2 : Saturate  UpperLimit=707  LowerLimit=-707
  Saturation3 : Saturate  UpperLimit=1418  LowerLimit=-1418
  Saturation4 : Saturate  UpperLimit=250  LowerLimit=-250
  term1 : Terminator
  term2 : Terminator
  term3 : Terminator
  Efd : Outport  VectorParamsAs1DForOutWhenUnconnected=off
  wires:
  It/1 -> term3/1
  Vt/1 -> Low-Pass Filter (Discrete or Continuous)/1
  Vref/1 -> Add/1
  Ifd/1 -> term1/1
  Vstab/1 -> term2/1
  Saturation4/1 -> Efd/1
  Add/1 -> Saturation/1
  Low-Pass Filter (Discrete or Continuous)/1 -> Low-Pass Filter (Discrete or Continuous)1/1
  Low-Pass Filter (Discrete or Continuous)1/1 -> Saturation1/1
  Add1/1 -> Add/2
  Saturation1/1 -> Gain/1, Add1/1
  Filtered Derivative (Discrete or Continuous)/1 -> Low-Pass Filter (Discrete or Continuous)2/1
  Gain/1 -> Filtered Derivative (Discrete or Continuous)/1
  Low-Pass Filter (Discrete or Continuous)2/1 -> Saturation2/1
  Saturation2/1 -> Add1/2
  Saturation/1 -> Gain1/1
  Gain1/1 -> Add2/1, PID Controller/1
  PID Controller/1 -> Saturation3/1
  Saturation3/1 -> Add2/2
  Add2/1 -> Gain2/1
  Gain2/1 -> Saturation4/1

== system Model_DG_Synchronous_Generator/Synchronous_Generator/SG_Control/Exciter/DC1A ==
  Vref : Inport
  Vt : Inport  Port=2
  It : Inport  Port=3
  Ifd : Inport  Port=4
  Vstab : Inport  Port=5
  DC1A : spsDC1AExcitationSystemLib/DC1A Excitation System  Tr=20e-3  KaTa=[46 0.06]  VRminmax=[-0.9 1.0]  KfTf=[0.1 1]  TbTc=[0 0]  KeTe=[0.05 0.46]  Efd12=[3.1 2.3]  SeEfd12=[0.33 0.10]  v0=[1,1.42734]  TsBlock=-2
  term3 : Terminator
  term4 : Terminator
  Efd : Outport  VectorParamsAs1DForOutWhenUnconnected=off
  wires:
  Vref/1 -> DC1A/1
  Vt/1 -> DC1A/2
  Vstab/1 -> DC1A/3
  DC1A/1 -> Efd/1
  It/1 -> term3/1
  Ifd/1 -> term4/1

== system Model_DG_Synchronous_Generator/Synchronous_Generator/SG_Control/Exciter/DC2A ==
  Vref : Inport
  Vt : Inport  Port=2
  It : Inport  Port=3
  Ifd : Inport  Port=4
  Vstab : Inport  Port=5
  DC2A : spsDC2AExcitationSystemLib/DC2A Excitation System  Tr=20e-3  KaTa=[300 0.01]  VRminmax=[-4.9 4.95]  KfTf=[0.02 0.675]  TbTc=[0 0]  KeTe=[1 1.33]  Efd12=[3.05 2.29]  SeEfd12=[0.279 0.117]  v0=[1,1.42734]  TsBlock=-2
  term3 : Terminator
  term4 : Terminator
  Efd : Outport  VectorParamsAs1DForOutWhenUnconnected=off
  wires:
  Vref/1 -> DC2A/1
  Vt/1 -> DC2A/2
  Vstab/1 -> DC2A/3
  DC2A/1 -> Efd/1
  It/1 -> term3/1
  Ifd/1 -> term4/1

== system Model_DG_Synchronous_Generator/Synchronous_Generator/SG_Control/Exciter/ST1A ==
  Vref : Inport
  Vt : Inport  Port=2
  It : Inport  Port=3
  Ifd : Inport  Port=4
  Vstab : Inport  Port=5
  ST1A : spsST1AExcitationSystemLib/ST1A Excitation System  Tr=20e-3  KaTa=[210 0.001]  VIminmax=[-999 999]  VAminmax=[-999 999]  VRminmax=[-6.0 6.43]  KfTf=[0.001 1]  TbTc=[1 1 0 0]  KLR=4.54  ILR=4.4  Kc=0.038  v0=[1,1.42734]  TsBlock=-2
  term3 : Terminator
  Efd : Outport  VectorParamsAs1DForOutWhenUnconnected=off
  wires:
  Vref/1 -> ST1A/1
  Vt/1 -> ST1A/2
  Ifd/1 -> ST1A/3
  Vstab/1 -> ST1A/4
  ST1A/1 -> Efd/1
  It/1 -> term3/1

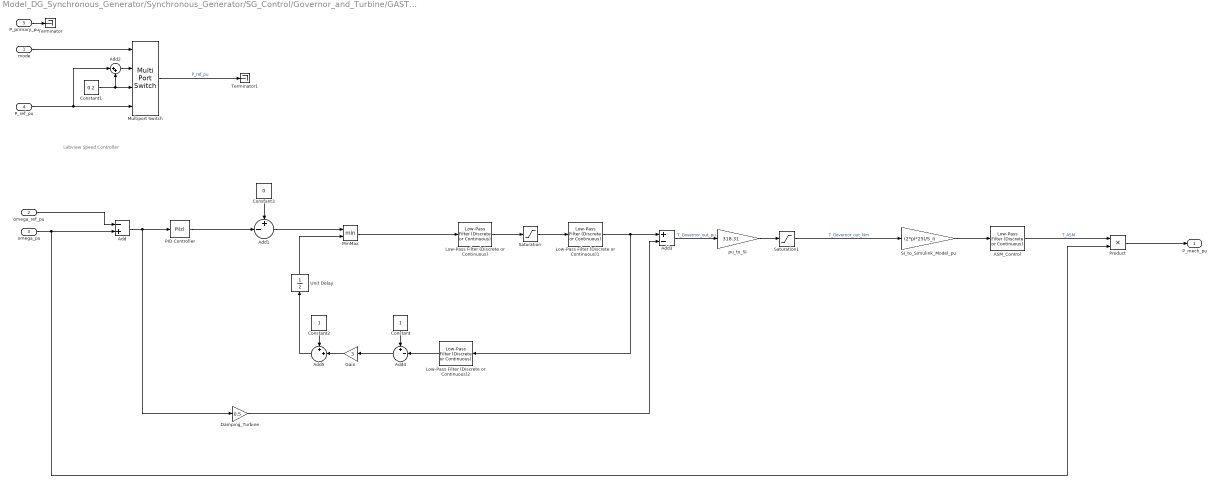
== system Model_DG_Synchronous_Generator/Synchronous_Generator/SG_Control/Governor_and_Turbine/GAST_SyncGen_Testbench_Huettenstrasse ==
  note: Labview Speed Controller
  mode : Inport
  omega_ref_pu : Inport  Port=2
  omega_pu : Inport  Port=3
  P_ref_pu : Inport  Port=4
  P_primary_pu : Inport  Port=5
  ASM_Control : eeGeneralControl/Low-Pass Filter (Discrete or Continuous)  K=0.9  T=0.02  B=inf  A=-inf  init_option=Inherited from block input  x0=0  Ts=-1
  Add : Sum  Inputs=-+
  Add1 : Sum  Inputs=+-|
  Add2 : Sum  Inputs=|++
  Add3 : Sum  Inputs=+-
  Add4 : Sum  Inputs=+-|
  Add5 : Sum  Inputs=++|
  Constant : Constant
  Constant1 : Constant  Value=0.2
  Constant2 : Constant
  Constant3 : Constant  Value=0
  Damping_Turbine : Gain  Gain=0.5
  Gain : Gain  Gain=3
  Low-Pass Filter (Discrete or Continuous) : eeGeneralControl/Low-Pass Filter (Discrete or Continuous)  K=1  T=0.03  B=inf  A=-inf  init_option=Inherited from block input  x0=0  Ts=-1
  Low-Pass Filter (Discrete or Continuous)1 : eeGeneralControl/Low-Pass Filter (Discrete or Continuous)  K=1  T=0.1  B=inf  A=-inf  init_option=Inherited from block input  x0=0  Ts=-1
  Low-Pass Filter (Discrete or Continuous)2 : eeGeneralControl/Low-Pass Filter (Discrete or Continuous)  K=1  T=2  B=inf  A=-inf  init_option=Inherited from block input  x0=0  Ts=-1
  MinMax : MinMax  Inputs=2
  Multiport Switch : MultiPortSwitch  DataPortOrder=Zero-based contiguous  zeroidx=on  SaturateOnIntegerOverflow=off  InputSameDT=off
  PID Controller : slpidlib/PID Controller  Controller=PI  Form=Parallel  TimeDomain=Discrete-time  UseExternalTs=off  SampleTime=-1  IntegratorMethod=Forward Euler  FilterMethod=Forward Euler  ControllerParametersSource=internal  P=10  I=16.67  UseKiTs=off  D=0  N=100  UseFilter=on  TunerSelectOption=Transfer Function Based (PID Tuner App)  InitialConditionSource=internal  InitialConditionForIntegrator=0  InitialConditionForFilter=0  DifferentiatorICPrevScaledInput=0  ExternalReset=none  TrackingMode=off  Kt=1  LimitOutput=off  SatLimitsSource=internal  UpperSaturationLimit=inf  LowerSaturationLimit=-inf  LinearizeAsGain=on  AntiWindupMode=none  Kb=1  LimitIntegrator=off  UpperIntegratorSaturationLimit=inf  LowerIntegratorSaturationLimit=-inf  POutMin=[]  POutMax=[]  IOutMin=[]  IOutMax=[]  DOutMin=[]  DOutMax=[]  NOutMin=[]  NOutMax=[]  SumOutMin=[]  SumOutMax=[]  SaturationOutMin=[]  SaturationOutMax=[]  PParamMin=[]  PParamMax=[]  IParamMin=[]  IParamMax=[]  DParamMin=[]  DParamMax=[]  NParamMin=[]  NParamMax=[]  KbParamMin=[]  KbParamMax=[]  KtParamMin=[]  KtParamMax=[]  KbOutMin=[]  KbOutMax=[]  KtOutMin=[]  KtOutMax=[]  IntegratorOutMin=[]  IntegratorOutMax=[]  FilterOutMin=[]  FilterOutMax=[]  SumI1OutMin=[]  SumI1OutMax=[]  SumI2OutMin=[]  SumI2OutMax=[]  SumI3OutMin=[]  SumI3OutMax=[]  SumI4OutMin=[]  SumI4OutMax=[]  SumDOutMin=[]  SumDOutMax=[]  DifferentiatorOutMin=[]  DifferentiatorOutMax=[]  FilterDiffOutCoefMin=[]  FilterDiffOutCoefMax=[]  ReciprocalOutMin=[]  ReciprocalOutMax=[]  SumDenOutMin=[]  SumDenOutMax=[]  SumNumOutMin=[]  SumNumOutMax=[]  DivideOutMin=[]  DivideOutMax=[]  UdiffTsProdOutMin=[]  UdiffTsProdOutMax=[]  NTsProdOutMin=[]  NTsProdOutMax=[]  UintegralTsProdOutMin=[]  UintegralTsProdOutMax=[]  UngainTsProdOutMin=[]  UngainTsProdOutMax=[]  ClampingZeroOutDataTypeStr=Inherit: Inherit via back propagation  ClampingZeroOutMin=[]  ClampingZeroOutMax=[]  FilterDenConstantOutDataTypeStr=Inherit: Inherit via back propagation  FilterDenConstantOutMin=[]  FilterDenConstantOutMax=[]  PCopyOutDataTypeStr=Inherit: Inherit via back propagation  PCopyOutMin=[]  PCopyOutMax=[]  NCopyOutDataTypeStr=Inherit: Inherit via back propagation  NCopyOutMin=[]  NCopyOutMax=[]  IntegratorContinuousStateAttributes=''  IntegratorStateMustResolveToSignalObject=off  IntegratorRTWStateStorageClass=Auto  FilterContinuousStateAttributes=''  FilterStateMustResolveToSignalObject=off  FilterRTWStateStorageClass=Auto  ParallelPVariant=InternalParameters  IdealPVariant=Disabled  IVariant=InternalParameters  DVariant=Disabled  IntegratorVariant=Discrete  SatVariant=Disabled  AWVariant=Passthrough  PCopyVariant=Disabled  TRVariant=Disabled  FdbkBlocksVariant=Forward  IdealPFdbkVariant=Disabled  SatFdbkVariant=Disabled  DerivativeFilterVariant=Disabled  NVariant=Disabled  NCopyVariant=Disabled_SignalSpec  FilterICVariant=Disabled  IntegratorICVariant=InternalICs  ExternalResetVariant=Disabled  TRSumVariant=Passthrough  SumFdbkVariant=Disabled  SumVariant=Sum_PI  TsampFilterVariant=InternalTs  TsampNgainVariant=Passthrough  TsampIntegralVariant=Passthrough  ExternalSaturationOutDataTypeStr=Inherit: Same as second input
  Product : Product  Inputs=**
  SI_to_Simulink_Model_pu : Gain  Gain=(2*pi*25)/S_n
  Saturation : Saturate  UpperLimit=1  LowerLimit=0
  Saturation1 : Saturate  UpperLimit=400  LowerLimit=-150
  Terminator : Terminator
  Terminator1 : Terminator
  Unit Delay : UnitDelay  InitialCondition=1  SampleTime=-1  HasFrameUpgradeWarning=on
  pu_to_SI : Gain  Gain=318.31
  P_mech_pu : Outport
  wires:
  Add2/1 -> Multiport Switch/2
  Constant1/1 -> Add2/2, Multiport Switch/3
  Multiport Switch/1 -> Terminator1/1  "P_ref_pu"
  mode/1 -> Multiport Switch/1
  P_ref_pu/1 -> Add2/1, Multiport Switch/4
  Add/1 -> Damping_Turbine/1, PID Controller/1
  omega_ref_pu/1 -> Add/1
  Add1/1 -> MinMax/1
  PID Controller/1 -> Add1/2
  Low-Pass Filter (Discrete or Continuous)/1 -> Saturation/1
  Saturation/1 -> Low-Pass Filter (Discrete or Continuous)1/1
  P_primary_pu/1 -> Terminator/1
  Low-Pass Filter (Discrete or Continuous)1/1 -> Low-Pass Filter (Discrete or Continuous)2/1, Add3/1
  Damping_Turbine/1 -> Add3/2
  Add3/1 -> pu_to_SI/1  "T_Governor_out_pu"
  MinMax/1 -> Low-Pass Filter (Discrete or Continuous)/1
  Low-Pass Filter (Discrete or Continuous)2/1 -> Add4/2
  Constant/1 -> Add4/1
  Add4/1 -> Gain/1
  Gain/1 -> Add5/2
  Constant2/1 -> Add5/1
  Add5/1 -> Unit Delay/1
  Unit Delay/1 -> MinMax/2
  Product/1 -> P_mech_pu/1
  omega_pu/1 -> Add/2, Product/2
  Constant3/1 -> Add1/1
  ASM_Control/1 -> Product/1  "T_ASM"
  pu_to_SI/1 -> Saturation1/1
  Saturation1/1 -> SI_to_Simulink_Model_pu/1  "T_Governor_out_Nm"
  SI_to_Simulink_Model_pu/1 -> ASM_Control/1

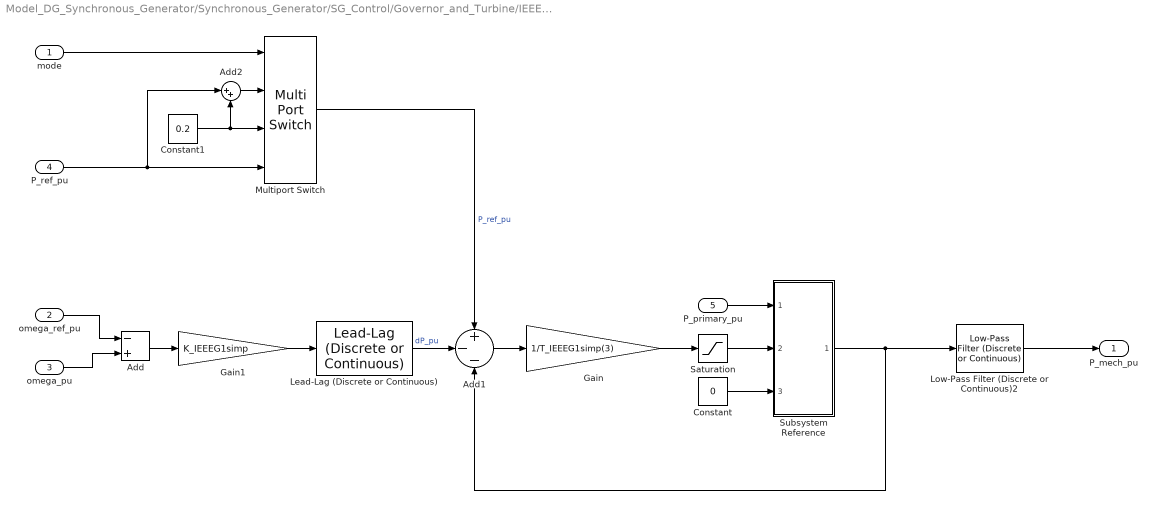
== system Model_DG_Synchronous_Generator/Synchronous_Generator/SG_Control/Governor_and_Turbine/IEEEG1_simplified ==
  mode : Inport
  omega_ref_pu : Inport  Port=2
  omega_pu : Inport  Port=3
  P_ref_pu : Inport  Port=4
  P_primary_pu : Inport  Port=5
  Add : Sum  Inputs=-+
  Add1 : Sum  Inputs=+--
  Add2 : Sum  Inputs=|++
  Constant : Constant  Value=0
  Constant1 : Constant  Value=0.2
  Gain : Gain  Gain=1/T_IEEEG1simp(3)
  Gain1 : Gain  Gain=K_IEEEG1simp
  Lead-Lag (Discrete or Continuous) : eeGeneralControl/Lead-Lag (Discrete or Continuous)  T1=T_IEEEG1simp(2)  T2=T_IEEEG1simp(1)  B=inf  A=-inf  init_option=Inherited from block input  x0=0  Ts=-1
  Low-Pass Filter (Discrete or Continuous)2 : eeGeneralControl/Low-Pass Filter (Discrete or Continuous)  K=1  T=T_IEEEG1simp(4)  B=inf  A=-inf  init_option=Inherited from block input  x0=0  Ts=-1
  Multiport Switch : MultiPortSwitch  DataPortOrder=Zero-based contiguous  zeroidx=on  SaturateOnIntegerOverflow=off  InputSameDT=off
  Saturation : Saturate  UpperLimit=dP_maxmin_IEEEG1simp(1)  LowerLimit=dP_maxmin_IEEEG1simp(2)
  Subsystem Reference : Subsystem  ReferencedSubsystem=Integrator_dyn_sat  initValue=0  T_s=-1
  P_mech_pu : Outport
  wires:
  P_ref_pu/1 -> Add2/1, Multiport Switch/4
  Low-Pass Filter (Discrete or Continuous)2/1 -> P_mech_pu/1
  Saturation/1 -> Subsystem Reference/2
  Gain/1 -> Saturation/1
  Subsystem Reference/1 -> Add1/3, Low-Pass Filter (Discrete or Continuous)2/1
  Add1/1 -> Gain/1
  omega_ref_pu/1 -> Add/1
  omega_pu/1 -> Add/2
  P_primary_pu/1 -> Subsystem Reference/1
  Constant/1 -> Subsystem Reference/3
  Add/1 -> Gain1/1
  Gain1/1 -> Lead-Lag (Discrete or Continuous)/1
  Lead-Lag (Discrete or Continuous)/1 -> Add1/2  "dP_pu"
  mode/1 -> Multiport Switch/1
  Multiport Switch/1 -> Add1/1  "P_ref_pu"
  Constant1/1 -> Add2/2, Multiport Switch/3
  Add2/1 -> Multiport Switch/2

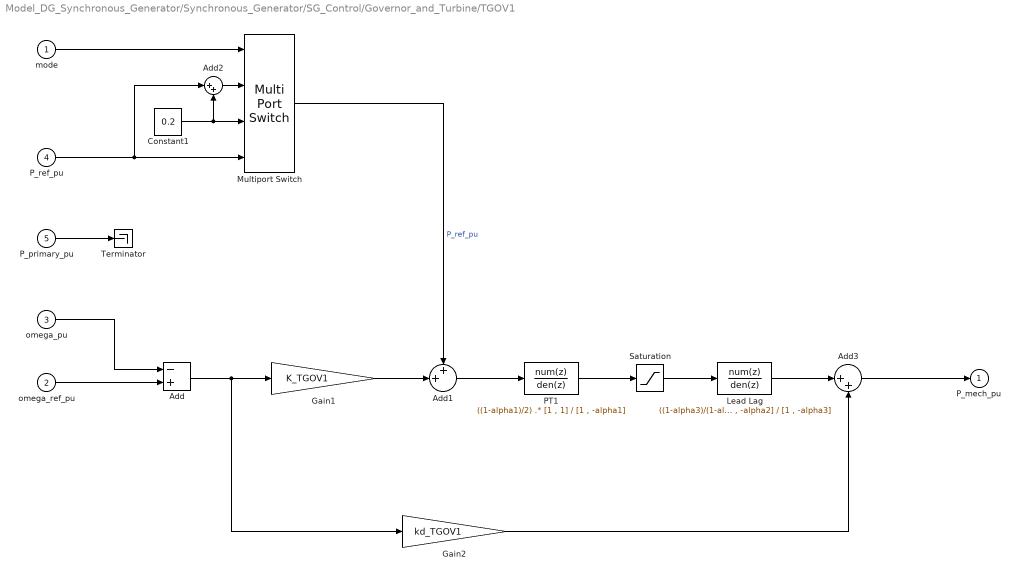
== system Model_DG_Synchronous_Generator/Synchronous_Generator/SG_Control/Governor_and_Turbine/TGOV1 ==
  mode : Inport
  omega_ref_pu : Inport  Port=2
  omega_pu : Inport  Port=3
  P_ref_pu : Inport  Port=4
  P_primary_pu : Inport  Port=5
  Add : Sum  Inputs=-+
  Add1 : Sum  Inputs=++|
  Add2 : Sum  Inputs=|++
  Add3 : Sum  Inputs=|++
  Constant1 : Constant  Value=0.2
  Gain1 : Gain  Gain=K_TGOV1
  Gain2 : Gain  Gain=kd_TGOV1
  Lead Lag : DiscreteTransferFcn  Numerator=((1-alpha3)/(1-alpha2)) .* [1 , -alpha2]  Denominator=[1 , -alpha3]
  Multiport Switch : MultiPortSwitch  DataPortOrder=Zero-based contiguous  zeroidx=on  SaturateOnIntegerOverflow=off  InputSameDT=off
  PT1 : DiscreteTransferFcn  Numerator=((1-alpha1)/2) .* [1 , 1]  Denominator=[1 , -alpha1]
  Saturation : Saturate  UpperLimit=1  LowerLimit=0
  Terminator : Terminator
  P_mech_pu : Outport
  wires:
  Multiport Switch/1 -> Add1/1  "P_ref_pu"
  Add2/1 -> Multiport Switch/2
  mode/1 -> Multiport Switch/1
  Constant1/1 -> Add2/2, Multiport Switch/3
  P_ref_pu/1 -> Add2/1, Multiport Switch/4
  Add/1 -> Gain2/1, Gain1/1
  omega_ref_pu/1 -> Add/2
  omega_pu/1 -> Add/1
  Gain1/1 -> Add1/2
  P_primary_pu/1 -> Terminator/1
  Add1/1 -> PT1/1
  PT1/1 -> Saturation/1
  Saturation/1 -> Lead Lag/1
  Lead Lag/1 -> Add3/1
  Gain2/1 -> Add3/2
  Add3/1 -> P_mech_pu/1
